simulink model "Main"  (R2023b)
settings: Solver=ode45  StartTime=0.0  StopTime=10.0  RelTol=1e-3  EnableMultiTasking=on
libraries: simulink x2
settings Model: Creator=Mojtaba  LastModifiedBy=Mojtaba
settings SolverCC: AlgebraicLoopSolver=TrustRegion
settings DataIOCC: LimitDataPoints=on  SaveFormat=Array  ReturnWorkspaceOutputs=off
settings OptimizationCC: LifeSpan=inf
settings DebuggingCC: UnderspecifiedInitializationDetection=Classic  MergeDetectMultiDrivingBlocksExec=none  SolverPrmCheckMsg=warning  UnconnectedInputMsg=warning  UnconnectedOutputMsg=warning  UnconnectedLineMsg=warning  StateNameClashWarn=warning  SFUnexpectedBacktrackingDiag=warning  SFNoUnconditionalDefaultTransitionDiag=warning  SFExecutionAtInitializationDiag=none  ArithmeticOperatorsInVariantConditions=warning
settings HardwareCC: ProdBitPerPointer=32  ProdBitPerSizeT=32  ProdBitPerPtrDiffT=32  ProdLargestAtomicFloat=None  ProdIntDivRoundTo=Undefined  ProdEndianess=Unspecified  ProdWordSize=32  ProdHWDeviceType=32-bit Generic
settings ModelReferenceCC: PropagateSignalLabelsOutOfModel=off
settings SFSimCC: SimUseLocalCustomCode=off  CustomCodeUndefinedFunction=UseInterfaceOnly
settings RTWCC: RTWUseLocalCustomCode=off
settings CodeAppCC: StateflowObjectComments=on
settings GRTTargetCC: TargetLangStandard=C89/C90 (ANSI)
settings ConfigComp: CovMetricSettings=dw  CovSaveCumulativeToWorkspaceVar=on  CovSaveSingleToWorkspaceVar=on  CovExternalEMLEnable=off

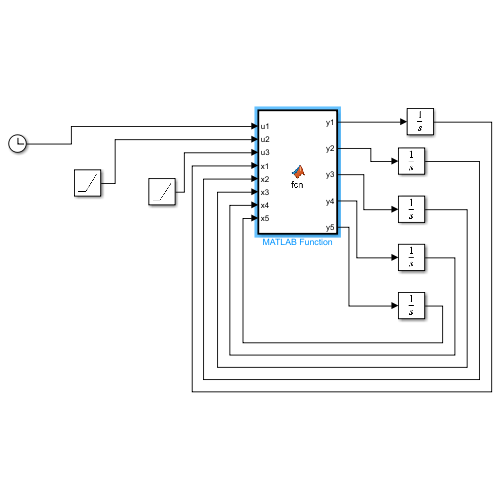
[thumbnail: Simulink's stored preview of the top-level diagram]
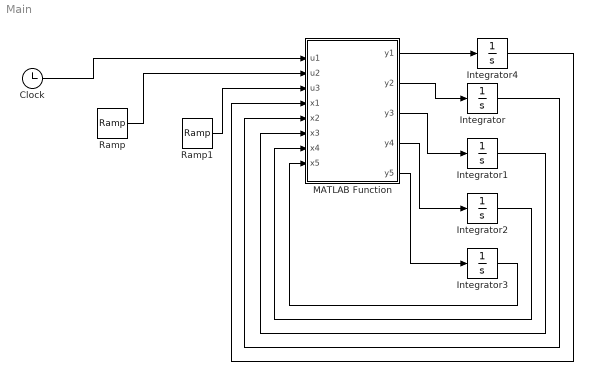
== system Main ==
  Clock : Clock
  Integrator{,1..4} (5 alike) : Integrator
  MATLAB Function : MATLAB Function  TreatAsAtomicUnit=on
  Ramp : simulink/Sources/Ramp  slope=1  start=0  InitialOutput=0
  Ramp1 : simulink/Sources/Ramp  slope=1  start=0  InitialOutput=0
  wires:
  Clock/1 -> MATLAB Function/1(u1)
  Ramp/1 -> MATLAB Function/2(u2)
  Ramp1/1 -> MATLAB Function/3(u3)
  MATLAB Function/1(y1) -> Integrator4/1
  MATLAB Function/2(y2) -> Integrator/1
  MATLAB Function/3(y3) -> Integrator1/1
  MATLAB Function/4(y4) -> Integrator2/1
  MATLAB Function/5(y5) -> Integrator3/1
  Integrator3/1 -> MATLAB Function/8(x5)
  Integrator2/1 -> MATLAB Function/7(x4)
  Integrator1/1 -> MATLAB Function/6(x3)
  Integrator/1 -> MATLAB Function/5(x2)
  Integrator4/1 -> MATLAB Function/4(x1)

== matlab function Main/MATLAB Function ==
  data: u1 input; y1 output; u2 input; u3 input; x1 input; x2 input; x3 input; x4 input; x5 input; y2 output; y3 output; y4 output; y5 output
function [y1,y2,y3,y4,y5] = fcn(u1,u2,u3,x1,x2,x3,x4,x5)
%% Ct  CdotT
Rs=1;
% RM=0.005;
% RA=0.001;
Rc=0.0398;
CR=4.4;
Cs=1.33;
CA=0.08;
Ls=0.0005;
Emax=2;
Emin=0.06;   %%%%%%
HR=1; 
%%
tc=60/HR;
Tmax=0.2+.15*tc;
tn=u1/Tmax;
s1=1.55*(((10*tn)/7)^1.9);
s2=1+(((10*tn)/7)^1.9);
s3=1+(tn/1.17)^21.9;
En=s1/(s2*s3);
E=(Emax-Emin)*En+Emin;
Ct=1/E;
t=u1;
CdotT=((0.88715838509316770186335403726708*(0.15527950310559006211180124223602*t)^(14/5))/(((0.15527950310559006211180124223602*t)^(19/10) + 1.0)^2*((0.092902266815310293571163136380528*t)^(219/10) + 1.0)) - (0.88715838509316770186335403726708*(0.15527950310559006211180124223602*t)^(9/10))/(((0.15527950310559006211180124223602*t)^(19/10) + 1.0)*((0.092902266815310293571163136380528*t)^(219/10) + 1.0)) + (6.1179208472686733556298773690078*(0.15527950310559006211180124223602*t)^(19/10)*(0.092902266815310293571163136380528*t)^(209/10))/(((0.15527950310559006211180124223602*t)^(19/10) + 1.0)*((0.092902266815310293571163136380528*t)^(219/10) + 1.0)^2))/((3.007*(0.15527950310559006211180124223602*t)^(19/10))/(((0.15527950310559006211180124223602*t)^(19/10) + 1.0)*((0.092902266815310293571163136380528*t)^(219/10) + 1.0)) + 0.06)^2;

a11=-CdotT*E;
A=[a11 0 0 0 0
    0 -1/(Rs*CR) 1/(Rs*CR) 0 0
    0 1/(Rs*Cs) 1/(Rs*Cs) 0 1/Cs
    0 0 0 0 1/CA
    0 0 -1/Ls 1/Ls -Rc/Ls];
B=[E -E
   -1/CR 0
    0 0
    0 1/CA
    0 0];
% C=eye(siz(A,1));
% D=[];
% sys1=ss(A,B,C,D);
% [yo,~,~]=lsim(sys1,[u2;u3],u1);+B*[u2;u3]
dx=A*[x1;x2;x3;x4;x5]+B*[u2;u3];
y1 =dx(1);
y2 =dx(2);
y3 =dx(3);
y4 =dx(4);
y5 =dx(5);
